simulink model "practica6_simulink"  (R2026a)
settings: Solver=VariableStepAuto  StopTime=0.005
InitFcn:
  | l = 2e-3;
  | r = 10;
  | c = 10e-6;
  | uin = 32;
  | f = 100e3;
  | d = 0.4;
settings Model: Creator=dante  LastModifiedBy=dante

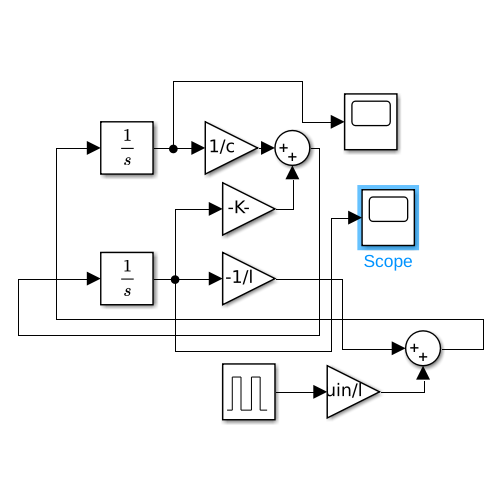
[thumbnail: Simulink's stored preview of the top-level diagram]
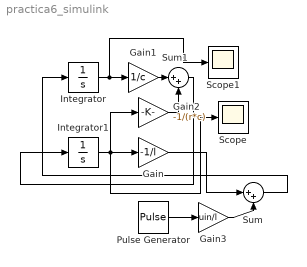
== system practica6_simulink ==
  Gain : Gain  Gain=-1/l
  Gain1 : Gain  Gain=1/c
  Gain2 : Gain  Gain=-1/(r*c)
  Gain3 : Gain  Gain=uin/l
  Integrator : Integrator
  Integrator1 : Integrator
  Pulse Generator : DiscretePulseGenerator  PulseType=Time based  Period=1/f  PulseWidth=d * 100
  Scope : Scope
      settings: ActiveDisplayYMinimum=-1.6690763206549943  ActiveDisplayYMaximum=15.021686885894953
  Scope1 : Scope
      settings: ActiveDisplayYMinimum=-0.17312047082165338  ActiveDisplayYMaximum=1.5580842373948807
  Sum : Sum  Inputs=|++
  Sum1 : Sum  Inputs=|++
  wires:
  Pulse Generator/1 -> Gain3/1
  Gain3/1 -> Sum/2
  Integrator1/1 -> Scope/1, Gain2/1, Gain/1
  Gain/1 -> Sum/1
  Sum/1 -> Integrator/1
  Integrator/1 -> Scope1/1, Gain1/1
  Gain1/1 -> Sum1/1
  Gain2/1 -> Sum1/2
  Sum1/1 -> Integrator1/1
